simulink model "unit_load_serial_rt"  (R2026b)
settings: Solver=FixedStepAuto  StopTime=inf  FixedStep=0.01
libraries: Lnx_ZK560103_Lib x2, simulink x1
settings Model: Creator=Administrator  LastModifiedBy=gao
settings OptimizationCC: BlockReduction=off  ReuseModelBlockBuffer=off
settings HardwareCC: ProdHWDeviceType=Intel->x86-64 (Linux 64)
settings RTWCC: SystemTargetFile=links_rtlnx_grt.tlc  TemplateMakefile=links_rtlnx_grt.tmf
settings STFCustomTargetCC: CombineOutputUpdateFcns=on  GRTInterface=off  SystemTargetFile=links_rtlnx_grt.tlc
settings GRTTargetCC: CPPClassGenCompliant=off  CompOptLevelCompliant=off  ConcurrentExecutionCompliant=off  MatFileLogging=off  ParMdlRefBuildCompliant=off  RTWCAPIParams=on  RTWCAPIRootIO=on  RTWCAPISignals=on

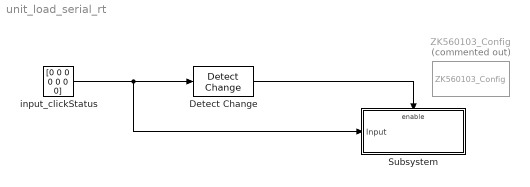
== system unit_load_serial_rt ==
  Detect Change : simulink/Logic and Bit Operations/Detect Change  vinit=[0 0 0 0 0 0 0]  OutDataTypeStr=boolean
  Subsystem : Subsystem
  ZK560103_Config : Lnx_ZK560103_Lib/ZK560103_Config  Commented=on  BoardOrder=0  PortOrder=3  BaudRate=9600  Parity=0(NO PARITY)  DataBits=8  StopBits=1  mode=RS232  SampleTime=-1
      settings: SourceProductName=Links_LnxLib
  input_clickStatus : Constant  Value=[0 0 0 0 0 0 0]  VectorParams1D=off
  wires:
  input_clickStatus/1 -> Subsystem/1(Input), Detect Change/1
  Detect Change/1 -> Subsystem/Enable

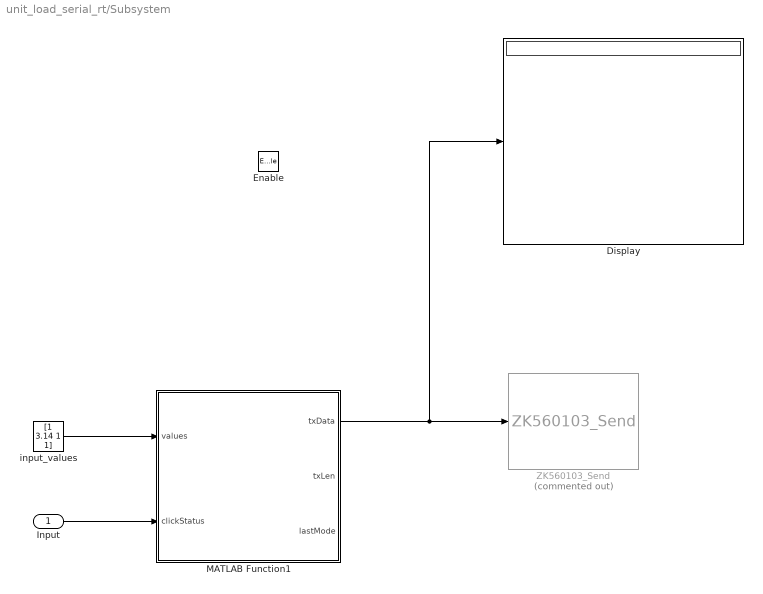
== system unit_load_serial_rt/Subsystem ==
  Input : Inport
  Enable : EnablePort
  Display : Display
      settings: Format=hex (Stored Integer)
  MATLAB Function1 : MATLAB Function  TreatAsAtomicUnit=on
  ZK560103_Send : Lnx_ZK560103_Lib/ZK560103_Send  Commented=on  BoardOrder=0  PortOrder=3  sendByteType=Auto  SampleTime=-1
      settings: SourceProductName=Links_LnxLib
  input_values : Constant  Value=[1 3.14 1 1]  VectorParams1D=off
  wires:
  MATLAB Function1/1(txData) -> ZK560103_Send/1, Display/1
  input_values/1 -> MATLAB Function1/1(values)
  Input/1 -> MATLAB Function1/2(clickStatus)

== matlab function unit_load_serial_rt/Subsystem/MATLAB Function1 ==
  data: values input; clickStatus input; txData output; txLen output; lastMode output
function [txData, txLen, lastMode] = unitload_cmd_gen(values, clickStatus)
    % values: [1x4] double 数组，分别对应 [电流设定, 电压设定, 电阻设定, 功率设定]
    % clickStatus: [1x7] double 数组，UI控件的拨动/点击状态
    %   1~4: 分别对应设置 电流、电压、电阻、功率 按钮 (发生变化即下发命令)
    %   5: Load 负载开关 (发生变化时下发最新状态)
    %   6: Short 短路开关 (发生变化时下发最新状态)
    %   7: Meas 测量查询按钮 (发生变化即下发命令)
    %
    % cmd: uint8 命令数组
    % len: 命令长度
    % lastMode: 当前停留的模式 (1=CURR, 2=VOLT, 3=RES, 4=POW) 用于UI指示灯显示

    MAX_LEN = 32;
    txData = zeros(1, MAX_LEN, 'uint8');
    txLen = 0;

    % 声明持久化变量 (相当于 Simulink 里的状态记忆)
    persistent prevClickStatus;
    persistent currentMode;

    % 初始状态赋初值 (系统刚上电时的第一拍执行)
    if isempty(prevClickStatus)
        prevClickStatus = zeros(1, 7);
    end
    if isempty(currentMode)
        currentMode = 1; % 默认停留在 1 (CURR模式)
    end

    LF = uint8(10); % 强制使用 ASCII 10 换行符
    cmd = uint8([]); % 用于存放最终的字节数组

    % --- 核心逻辑：检测哪个按钮的状态发生了变化 (边缘检测) ---
    diffStatus = clickStatus - prevClickStatus;
    changedIdx = 0;
    for k = 1:7
        if abs(diffStatus(k)) > 0
            changedIdx = k;
            break;
        end
    end


    % --- 根据发生变化的按钮，组装相应的命令 ---
    if changedIdx > 0
        switch changedIdx
            case 1 % 触发了“设置电流”
                currentMode = 1;
                cmd = [uint8('MODE CURR'), LF, uint8(sprintf('CURR %.4f',values(1))), LF];

            case 2 % 触发了“设置电压”
                currentMode = 2;
                cmd = [uint8('MODE VOLT'), LF,uint8(sprintf('VOLT %.4f',values(2))), LF];

            case 3 % 触发了“设置电阻”
                currentMode = 3;
                cmd = [uint8('MODE RES'), LF, uint8(sprintf('RES %.4f',values(3))), LF];

            case 4 % 触发了“设置功率”
                currentMode = 4;
                cmd = [uint8('MODE POW'), LF,uint8(sprintf('POW %.4f',values(4))), LF];

            case 5 % 触发了 Load 负载开关
                if clickStatus(5) > 0
                    cmd = [uint8('INP 1'), LF];
                else
                    cmd = [uint8('INP 0'), LF];
                end

            case 6 % 触发了 Short 开关
                if clickStatus(6) > 0
                    cmd = [uint8('INP:SHOR 1'), LF];
                else
                    cmd = [uint8('INP:SHOR 0'), LF];
                end

            case 7 % 触发了 Meas 测量
                cmd = [uint8('MEAS:REAL?'), LF];
        end
    end

    % --- 更新记忆状态，供下一个轮询周期对比 ---
    prevClickStatus = clickStatus;
    lastMode = currentMode;

    % --- 转换为输出的底层字节 ---
    txLen = double(numel(cmd));
    if txLen > MAX_LEN
        txLen = MAX_LEN; % 防止溢出
    end
    if txLen > 0
        txData(1:txLen) = cmd(1:txLen);
    end
end
